simulink model "HoverStateMachine"  (R2024a)
settings: Solver=VariableStepAuto  StartTime=0.0  StopTime=10.0  RelTol=1e-3
settings Model: Creator=joshkahn  LastModifiedBy=joshkahn

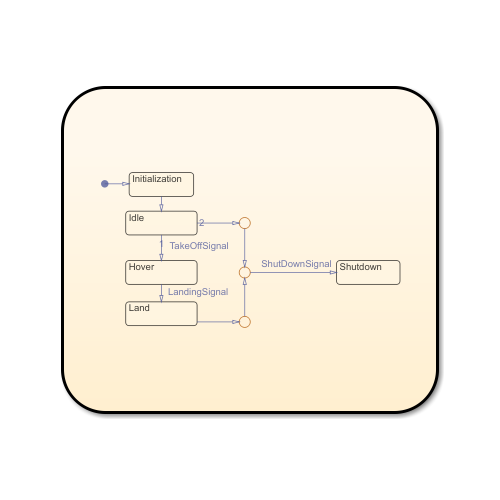
[thumbnail: Simulink's stored preview of the top-level diagram]
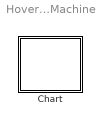
== system HoverStateMachine ==
  Chart : Stateflow chart  TreatAsAtomicUnit=on

== stateflow chart HoverStateMachine/Chart ==
  state Initialization
  state Idle
  state Hover
  state Shutdown
  state Land
  (default) -> Initialization
  Initialization -> Idle
  Idle -> (junction 18) [order 2]
  (junction 18) -> (junction 17)
  Idle -> Hover [order 1] : TakeOffSignal
  (junction 17) -> Shutdown : ShutDownSignal
  (junction 19) -> (junction 17)
  Hover -> Land : LandingSignal
  Land -> (junction 19)
